simulink model "DIGITAL_WATCH_STAGE4"  (R2026b)
settings: Solver=VariableStepAuto  StopTime=59
libraries: simulink_extras x7
settings Model: Creator=Trealer  LastModifiedBy=Trealer

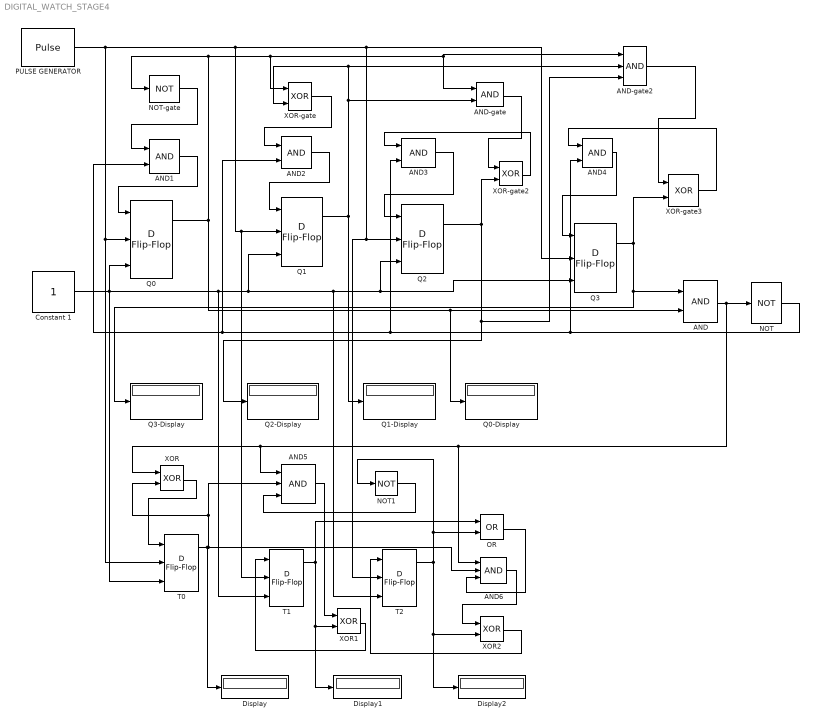
== system DIGITAL_WATCH_STAGE4 ==
  AND{,1..4} (5 alike) : Logic  IconShape=distinctive  AllPortsSameDT=off  OutDataTypeStr=boolean
  AND-gate : Logic  IconShape=distinctive  AllPortsSameDT=off  OutDataTypeStr=boolean
  AND-gate2 : Logic  Inputs=3  IconShape=distinctive  AllPortsSameDT=off  OutDataTypeStr=boolean
  AND5 : Logic  Inputs=3  IconShape=distinctive  AllPortsSameDT=off  OutDataTypeStr=boolean
  AND6 : Logic  Inputs=3  IconShape=distinctive  AllPortsSameDT=off  OutDataTypeStr=boolean
  Constant 1 : Constant
  Display : Display
  Display1 : Display
  Display2 : Display
  NOT : Logic  Operator=NOT  IconShape=distinctive  AllPortsSameDT=off  OutDataTypeStr=boolean
  NOT-gate : Logic  Operator=NOT  IconShape=distinctive  AllPortsSameDT=off  OutDataTypeStr=boolean
  NOT1 : Logic  Operator=NOT  IconShape=distinctive  AllPortsSameDT=off  OutDataTypeStr=boolean
  OR : Logic  Operator=OR  IconShape=distinctive  AllPortsSameDT=off  OutDataTypeStr=boolean
  PULSE GENERATOR : DiscretePulseGenerator  PulseType=Time based  Period=1  PulseWidth=50
  Q{0..3} (4 alike) : simulink_extras/Flip Flops/D Flip-Flop
  Q0-Display : Display
  Q1-Display : Display
  Q2-Display : Display
  Q3-Display : Display
  T0 : simulink_extras/Flip Flops/D Flip-Flop
  T1 : simulink_extras/Flip Flops/D Flip-Flop
  T2 : simulink_extras/Flip Flops/D Flip-Flop
  XOR : Logic  Operator=XOR  IconShape=distinctive  AllPortsSameDT=off  OutDataTypeStr=boolean
  XOR-gate : Logic  Operator=XOR  IconShape=distinctive  AllPortsSameDT=off  OutDataTypeStr=boolean
  XOR-gate2 : Logic  Operator=XOR  IconShape=distinctive  AllPortsSameDT=off  OutDataTypeStr=boolean
  XOR-gate3 : Logic  Operator=XOR  IconShape=distinctive  AllPortsSameDT=off  OutDataTypeStr=boolean
  XOR1 : Logic  Operator=XOR  IconShape=distinctive  AllPortsSameDT=off  OutDataTypeStr=boolean
  XOR2 : Logic  Operator=XOR  IconShape=distinctive  AllPortsSameDT=off  OutDataTypeStr=boolean
  wires:
  PULSE GENERATOR/1 -> Q3/2, T2/2, Q2/2, Q1/2, T1/2, Q0/2, T0/2
  Constant 1/1 -> T1/3, T2/3, Q3/3, Q2/3, Q1/3, Q0/3, T0/3
  Q0/1 -> AND-gate/1, AND-gate2/1, XOR-gate/1, NOT-gate/1, Q0-Display/1, AND/2
  Q1/1 -> AND-gate2/2, XOR-gate/2, AND-gate/2, Q1-Display/1
  AND-gate/1 -> XOR-gate2/1
  Q2/1 -> XOR-gate2/2, Q2-Display/1, AND-gate2/3
  AND-gate2/1 -> XOR-gate3/1
  Q3/1 -> XOR-gate3/2, Q3-Display/1, AND/1
  AND/1 -> AND6/1, AND5/1, XOR/1, NOT/1
  NOT-gate/1 -> AND1/1
  XOR-gate/1 -> AND2/1
  XOR-gate2/1 -> AND3/1
  XOR-gate3/1 -> AND4/1
  AND1/1 -> Q0/1
  AND2/1 -> Q1/1
  AND3/1 -> Q2/1
  AND4/1 -> Q3/1
  NOT/1 -> AND4/2, AND3/2, AND1/2, AND2/2
  T0/1 -> Display/1, AND5/2, XOR/2, AND6/2
  XOR/1 -> T0/1
  T2/1 -> Display2/1, XOR2/2, OR/2, NOT1/1
  NOT1/1 -> AND5/3
  AND5/1 -> XOR1/1
  T1/1 -> Display1/1, XOR1/2, OR/1
  OR/1 -> AND6/3
  AND6/1 -> XOR2/1
  XOR1/1 -> T1/1
  XOR2/1 -> T2/1
